simulink subsystem "GravityField"  (R2024b)
settings: Solver=VariableStepAuto  StartTime=0.0  StopTime=10.0  RelTol=1e-3
undefined symbols (not defined in the file): gravAtt, gravLaplace
settings Model: Creator=pierb  LastModifiedBy=pierb

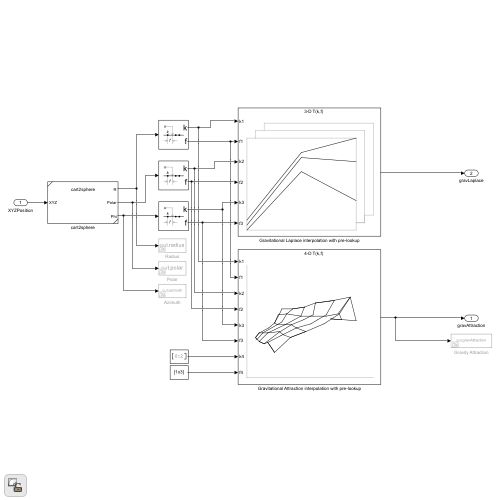
[thumbnail: Simulink's stored preview of the top-level diagram]
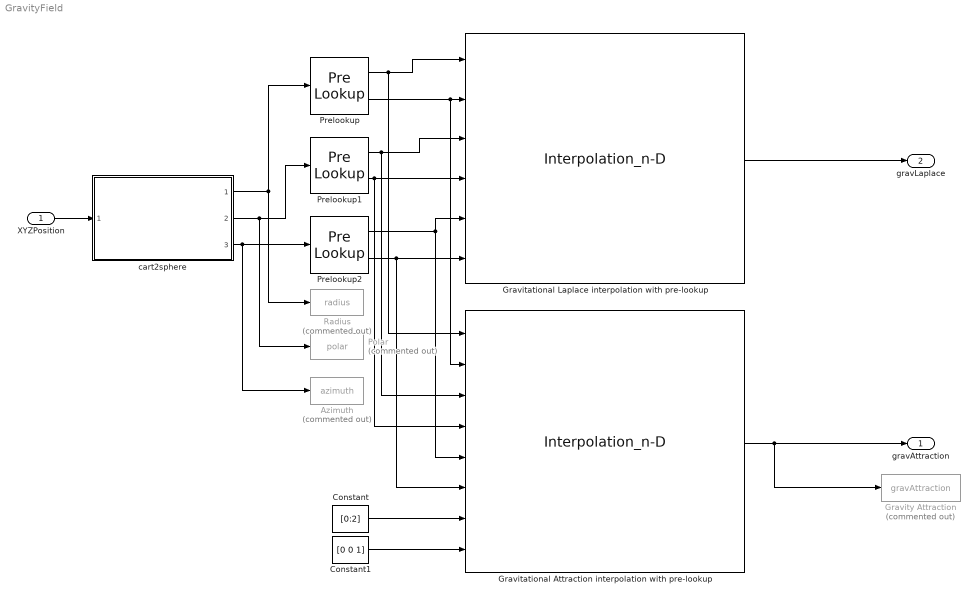
== system GravityField ==
  XYZPosition : Inport
  Azimuth : ToWorkspace  Commented=on  VariableName=azimuth  SampleTime=-1
  Constant : Constant  Value=[0:2]
  Constant1 : Constant  Value=[0 0 1]
  Gravitational Attraction interpolation with pre-lookup : Interpolation_n-D  NumberOfTableDimensions=4  Table=gravAtt  ExtrapMethod=Clip  InternalRulePriority=Speed  RndMeth=Simplest
      settings: InputPortMap=u0,u1,u2,u3,u4,u5,u6,u7
  Gravitational Laplace interpolation with pre-lookup : Interpolation_n-D  NumberOfTableDimensions=3  Table=gravLaplace  ExtrapMethod=Clip  InternalRulePriority=Speed  RndMeth=Simplest
      settings: InputPortMap=u0,u1,u2,u3,u4,u5
  Gravity Attraction : ToWorkspace  Commented=on  VariableName=gravAttraction  SaveFormat=Timeseries  SampleTime=-1
  Polar : ToWorkspace  Commented=on  VariableName=polar  SampleTime=-1
  Prelookup : PreLookup  BreakpointsData=environment.asteroidCoords.radius  BeginIndexSearchUsingPreviousIndexResult=on  ExtrapMethod=Linear  RndMeth=Simplest
  Prelookup1 : PreLookup  BreakpointsData=environment.asteroidCoords.polar  IndexSearchMethod=Linear search  BeginIndexSearchUsingPreviousIndexResult=on  DiagnosticForOutOfRangeInput=Warning  RndMeth=Simplest
  Prelookup2 : PreLookup  BreakpointsData=environment.asteroidCoords.azimuth  IndexSearchMethod=Linear search  BeginIndexSearchUsingPreviousIndexResult=on  RndMeth=Simplest
  Radius : ToWorkspace  Commented=on  VariableName=radius  SampleTime=-1
  cart2sphere : Subsystem  ReferencedSubsystem=cart2sphere
  gravAttraction : Outport
  gravLaplace : Outport  Port=2
  wires:
  XYZPosition/1 -> cart2sphere/1
  cart2sphere/3 -> Azimuth/1, Prelookup2/1
  cart2sphere/2 -> Polar/1, Prelookup1/1
  Prelookup1/1 -> Gravitational Attraction interpolation with pre-lookup/3, Gravitational Laplace interpolation with pre-lookup/3
  Prelookup/1 -> Gravitational Attraction interpolation with pre-lookup/1, Gravitational Laplace interpolation with pre-lookup/1
  Prelookup/2 -> Gravitational Laplace interpolation with pre-lookup/2, Gravitational Attraction interpolation with pre-lookup/2
  Prelookup1/2 -> Gravitational Laplace interpolation with pre-lookup/4, Gravitational Attraction interpolation with pre-lookup/4
  Prelookup2/1 -> Gravitational Attraction interpolation with pre-lookup/5, Gravitational Laplace interpolation with pre-lookup/5
  Prelookup2/2 -> Gravitational Attraction interpolation with pre-lookup/6, Gravitational Laplace interpolation with pre-lookup/6
  Constant/1 -> Gravitational Attraction interpolation with pre-lookup/7
  Constant1/1 -> Gravitational Attraction interpolation with pre-lookup/8
  Gravitational Laplace interpolation with pre-lookup/1 -> gravLaplace/1
  cart2sphere/1 -> Prelookup/1, Radius/1
  Gravitational Attraction interpolation with pre-lookup/1 -> gravAttraction/1, Gravity Attraction/1
